simulink model "bimanual_Diedrichsen"  (Simulink 8.1)
settings: Solver=ode4  SolverMode=SingleTasking  StartTime=0.0  StopTime=inf  FixedStep=0.0005  RelTol=1e-3
StartFcn:
  |  warndlg('Dexterit-E models cannot run under simulation. Please compile your model and run it from within Dexterit-E.');set_param(bdroot,'SimulationCommand','stop')
undefined symbols (not defined in the file or in its folder): slselsubs
libraries: Video x3, General x3, KINARM_EP_loads x3, KINARM_general x2, KINARM_loads x2, xpclib x1
(part 2 of 3)

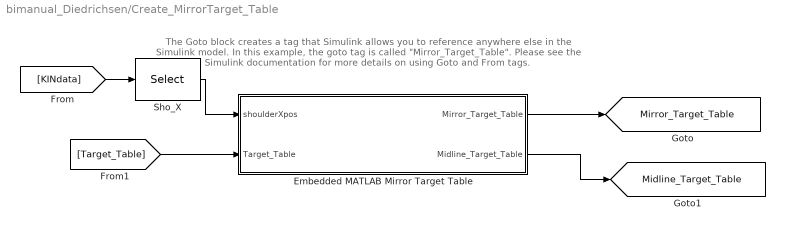
== system bimanual_Diedrichsen/Create_MirrorTarget_Table ==
  note: The Goto block creates a tag that Simulink allows you to reference anywhere else in the Simulink model.
      | In this example, the goto tag is called "Mirror_Target_Table".  Please see the Simulink documentation for more
      | details on using Goto and From tags.
  Embedded MATLAB Mirror Target Table : MATLAB Function  TreatAsAtomicUnit=on
  Sho_X : Selector  NumberOfDimensions=2  InputPortWidth=3  IndexOptions=Index vector (dialog),Index vector (dialog)  Indices=[1:2],[4]  OutputSizes=1
  tag scope: Midline_Target_Table=global, Mirror_Target_Table=global
  wires:
  [Target_Table] -> Embedded MATLAB Mirror Target Table/2(Target_Table)
  [KINdata] -> Sho_X/1
  Embedded MATLAB Mirror Target Table/1(Mirror_Target_Table) -> [Mirror_Target_Table]
  Sho_X/1 -> Embedded MATLAB Mirror Target Table/1(shoulderXpos)
  Embedded MATLAB Mirror Target Table/2(Midline_Target_Table) -> [Midline_Target_Table]

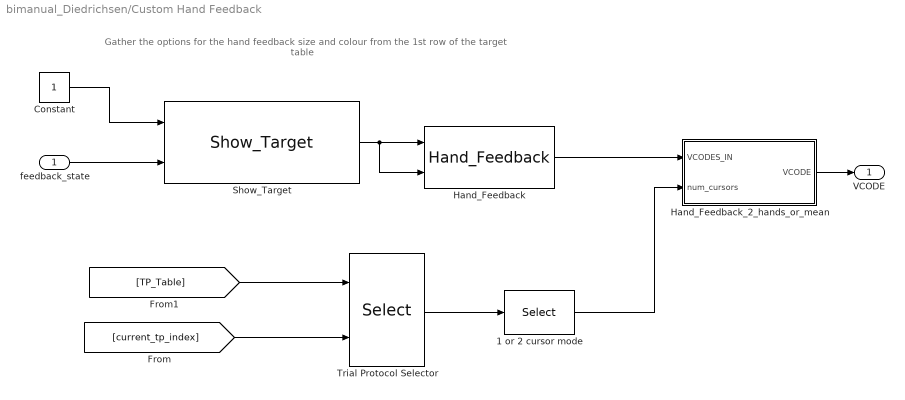
== system bimanual_Diedrichsen/Custom Hand Feedback ==
  note: Gather the options for the hand feedback size and colour from the 1st row of the target table
  "feedback_state " : Inport
  1 or 2 cursor mode : Selector  IndexOptions=Index vector (dialog)  Indices=4  OutputSizes=1
  Constant : Constant
  Hand_Feedback : KINARM_general/Hand_Feedback  feedback_cntl_src=style and status
  Hand_Feedback_2_hands_or_mean : Subsystem
  Show_Target : Video/Show_Target  target_type=Circle  num_states=4  attribcol1=[6 6 0 3]  attribcol2=[7 7 0 5]  attribcol3=[8 8 0 5]  attribcol4=[9 9 0 5]  attribcol5=[0 0 24 0]  stateindices_padding=[0 0 0 0 0 0 0;0 0 0 0 0 0 0;0 0 0 0 0 0 0;0 0 0 0 0 0 0;0 0 0 0 0 0 0]  source=dialog  opacity=100  target_display=Both subject and operator displays  num_col=4
  Trial Protocol Selector : Selector  NumberOfDimensions=2  InputPortWidth=3  IndexOptions=Index vector (port),Select all  Indices=1,-1  OutputSizes=1
  VCODE : Outport
  wires:
  "feedback_state "/1 -> Show_Target/2
  Constant/1 -> Show_Target/1
  Show_Target/1 -> Hand_Feedback/2, Hand_Feedback/1
  Trial Protocol Selector/1 -> 1 or 2 cursor mode/1
  [current_tp_index] -> Trial Protocol Selector/2
  [TP_Table] -> Trial Protocol Selector/1
  Hand_Feedback/1 -> Hand_Feedback_2_hands_or_mean/1(VCODES_IN)
  1 or 2 cursor mode/1 -> Hand_Feedback_2_hands_or_mean/2(num_cursors)
  Hand_Feedback_2_hands_or_mean/1(VCODE) -> VCODE/1

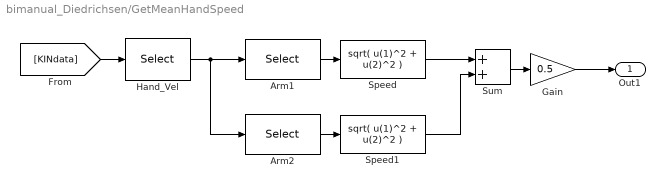
== system bimanual_Diedrichsen/GetMeanHandSpeed ==
  Arm1 : Selector  NumberOfDimensions=2  InputPortWidth=3  IndexOptions=Index vector (dialog),Select all  Indices=1,-1  OutputSizes=1
  Arm2 : Selector  NumberOfDimensions=2  InputPortWidth=3  IndexOptions=Index vector (dialog),Select all  Indices=2,-1  OutputSizes=1
  Gain : Gain  Gain=0.5
  Hand_Vel : Selector  NumberOfDimensions=2  InputPortWidth=3  IndexOptions=Select all,Index vector (dialog)  Indices=-1,[25,26]  OutputSizes=1
  Speed : Fcn  Expr=sqrt( u(1)^2 + u(2)^2 )
  Speed1 : Fcn  Expr=sqrt( u(1)^2 + u(2)^2 )
  Sum : Sum
  Out1 : Outport
  wires:
  Arm2/1 -> Speed1/1
  Sum/1 -> Gain/1
  Hand_Vel/1 -> Arm1/1, Arm2/1
  Arm1/1 -> Speed/1
  [KINdata] -> Hand_Vel/1
  Speed/1 -> Sum/1
  Speed1/1 -> Sum/2
  Gain/1 -> Out1/1

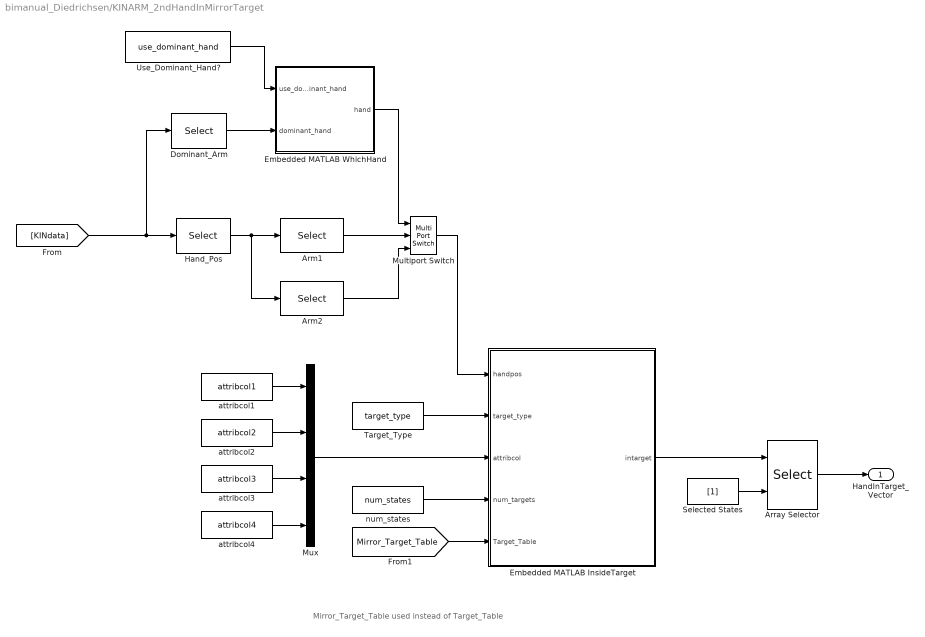
== system bimanual_Diedrichsen/KINARM_2ndHandInMirrorTarget ==
  note: Mirror_Target_Table used instead of Target_Table
  Arm1 : Selector  NumberOfDimensions=2  InputPortWidth=3  IndexOptions=Index vector (dialog),Select all  Indices=1,-1  OutputSizes=slselsubs([(-2),(-2)],1),slselsubs([(-2),(-2)],2)
  Arm2 : Selector  NumberOfDimensions=2  InputPortWidth=3  IndexOptions=Index vector (dialog),Select all  Indices=2,-1  OutputSizes=slselsubs([(-2),(-2)],1),slselsubs([(-2),(-2)],2)
  Array Selector : Selector  NumberOfDimensions=2  InputPortWidth=3  IndexOptions=Select all,Index vector (port)  Indices=-1,1  OutputSizes=slselsubs([(-2),(-2)],1),slselsubs([(-2),(-2)],2)
  Dominant_Arm : Selector  NumberOfDimensions=2  InputPortWidth=3  IndexOptions=Index vector (dialog),Index vector (dialog)  Indices=[3],[1]  OutputSizes=slselsubs([(-2),(-2)],1),slselsubs([(-2),(-2)],2)
  Embedded MATLAB InsideTarget : MATLAB Function  TreatAsAtomicUnit=on
  Embedded MATLAB WhichHand : MATLAB Function  TreatAsAtomicUnit=on
  Hand_Pos : Selector  NumberOfDimensions=2  InputPortWidth=3  IndexOptions=Select all,Index vector (dialog)  Indices=-1,[23,24]  OutputSizes=slselsubs([(-2),(-2)],1),slselsubs([(-2),(-2)],2)
  Multiport Switch : MultiPortSwitch  Inputs=2
  Mux : Mux
  Selected States : Constant  Value=[1]
  Target_Type : Constant  Value=target_type
  Use_Dominant_Hand? : Constant  Value=use_dominant_hand
  attribcol1 : Constant  Value=attribcol1
  attribcol2 : Constant  Value=attribcol2
  attribcol3 : Constant  Value=attribcol3
  attribcol4 : Constant  Value=attribcol4
  num_states : Constant  Value=num_states
  HandInTarget_Vector : Outport
  wires:
  Selected States/1 -> Array Selector/2
  num_states/1 -> Embedded MATLAB InsideTarget/4(num_targets)
  Mux/1 -> Embedded MATLAB InsideTarget/3(attribcol)
  attribcol4/1 -> Mux/4
  attribcol3/1 -> Mux/3
  attribcol2/1 -> Mux/2
  attribcol1/1 -> Mux/1
  Use_Dominant_Hand?/1 -> Embedded MATLAB WhichHand/1(use_dominant_hand)
  Embedded MATLAB WhichHand/1(hand) -> Multiport Switch/1
  Target_Type/1 -> Embedded MATLAB InsideTarget/2(target_type)
  Array Selector/1 -> HandInTarget_Vector/1
  [Mirror_Target_Table] -> Embedded MATLAB InsideTarget/5(Target_Table)
  Embedded MATLAB InsideTarget/1(intarget) -> Array Selector/1
  Multiport Switch/1 -> Embedded MATLAB InsideTarget/1(handpos)
  Arm2/1 -> Multiport Switch/3
  Arm1/1 -> Multiport Switch/2
  Dominant_Arm/1 -> Embedded MATLAB WhichHand/2(dominant_hand)
  Hand_Pos/1 -> Arm2/1, Arm1/1
  [KINdata] -> Dominant_Arm/1, Hand_Pos/1

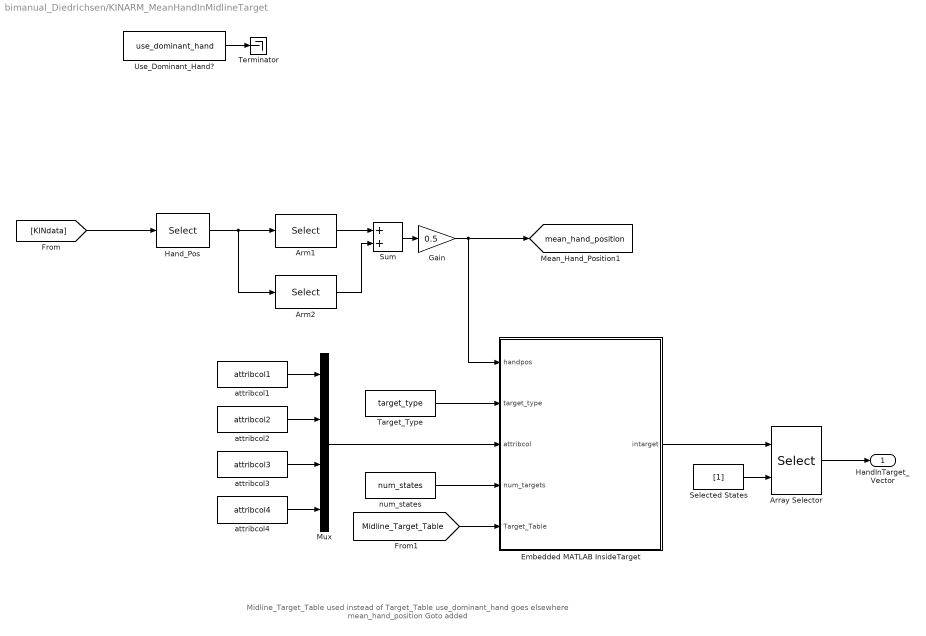
== system bimanual_Diedrichsen/KINARM_MeanHandInMidlineTarget ==
  note: Midline_Target_Table used instead of Target_Table
      | use_dominant_hand goes elsewhere
      | mean_hand_position Goto added
  Arm1 : Selector  NumberOfDimensions=2  InputPortWidth=3  IndexOptions=Index vector (dialog),Select all  Indices=1,-1  OutputSizes=1
  Arm2 : Selector  NumberOfDimensions=2  InputPortWidth=3  IndexOptions=Index vector (dialog),Select all  Indices=2,-1  OutputSizes=1
  Array Selector : Selector  NumberOfDimensions=2  InputPortWidth=3  IndexOptions=Select all,Index vector (port)  Indices=-1,1  OutputSizes=slselsubs([(-2),(-2)],1),slselsubs([(-2),(-2)],2)
  Embedded MATLAB InsideTarget : MATLAB Function  TreatAsAtomicUnit=on
  Gain : Gain  Gain=0.5
  Hand_Pos : Selector  NumberOfDimensions=2  InputPortWidth=3  IndexOptions=Select all,Index vector (dialog)  Indices=-1,[23,24]  OutputSizes=1
  Mux : Mux
  Selected States : Constant  Value=[1]
  Sum : Sum
  Target_Type : Constant  Value=target_type
  Terminator : Terminator
  Use_Dominant_Hand? : Constant  Value=use_dominant_hand
  attribcol1 : Constant  Value=attribcol1
  attribcol2 : Constant  Value=attribcol2
  attribcol3 : Constant  Value=attribcol3
  attribcol4 : Constant  Value=attribcol4
  num_states : Constant  Value=num_states
  HandInTarget_Vector : Outport
  tag scope: mean_hand_position=global
  wires:
  Selected States/1 -> Array Selector/2
  num_states/1 -> Embedded MATLAB InsideTarget/4(num_targets)
  Mux/1 -> Embedded MATLAB InsideTarget/3(attribcol)
  attribcol4/1 -> Mux/4
  attribcol3/1 -> Mux/3
  attribcol2/1 -> Mux/2
  attribcol1/1 -> Mux/1
  Target_Type/1 -> Embedded MATLAB InsideTarget/2(target_type)
  Array Selector/1 -> HandInTarget_Vector/1
  [Midline_Target_Table] -> Embedded MATLAB InsideTarget/5(Target_Table)
  Embedded MATLAB InsideTarget/1(intarget) -> Array Selector/1
  Gain/1 -> [mean_hand_position], Embedded MATLAB InsideTarget/1(handpos)
  Arm2/1 -> Sum/2
  Arm1/1 -> Sum/1
  Hand_Pos/1 -> Arm2/1, Arm1/1
  [KINdata] -> Hand_Pos/1
  Use_Dominant_Hand?/1 -> Terminator/1
  Sum/1 -> Gain/1

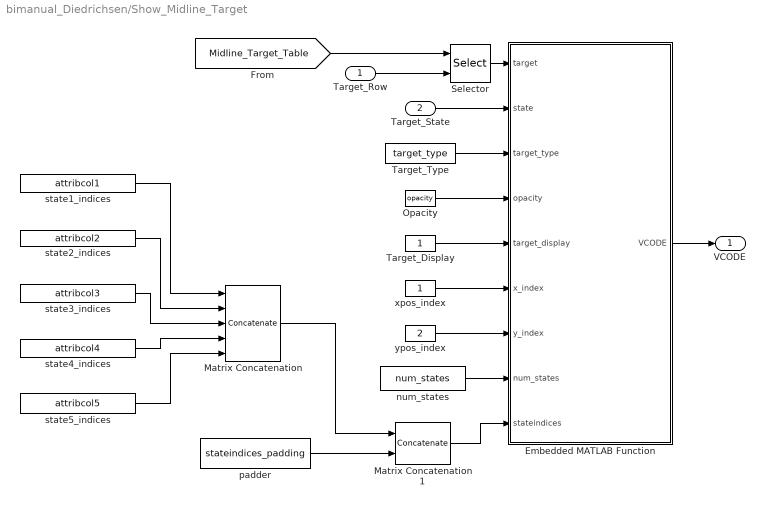
== system bimanual_Diedrichsen/Show_Midline_Target ==
  Target_Row : Inport
  Target_State : Inport  Port=2
  Embedded MATLAB Function : MATLAB Function  TreatAsAtomicUnit=on
  Matrix Concatenation : Concatenate  NumInputs=5  Mode=Multidimensional array
  Matrix Concatenation1 : Concatenate  Mode=Multidimensional array  ConcatenateDimension=2
  Opacity : Constant  Value=opacity
  Selector : Selector  NumberOfDimensions=2  InputPortWidth=3  IndexOptions=Index vector (port),Select all  Indices=1,-1  OutputSizes=slselsubs([(-2),(-2)],1),slselsubs([(-2),(-2)],2)
  Target_Display : Constant
  Target_Type : Constant  Value=target_type
  num_states : Constant  Value=num_states
  padder : Constant  Value=stateindices_padding
  state1_indices : Constant  Value=attribcol1  VectorParams1D=off
  state2_indices : Constant  Value=attribcol2  VectorParams1D=off
  state3_indices : Constant  Value=attribcol3  VectorParams1D=off
  state4_indices : Constant  Value=attribcol4  VectorParams1D=off
  state5_indices : Constant  Value=attribcol5  VectorParams1D=off
  xpos_index : Constant
  ypos_index : Constant  Value=2
  VCODE : Outport  PortDimensions=[1 70]
  wires:
  Target_Display/1 -> Embedded MATLAB Function/5(target_display)
  state2_indices/1 -> Matrix Concatenation/2
  state1_indices/1 -> Matrix Concatenation/1
  state5_indices/1 -> Matrix Concatenation/5
  state4_indices/1 -> Matrix Concatenation/4
  state3_indices/1 -> Matrix Concatenation/3
  Matrix Concatenation1/1 -> Embedded MATLAB Function/9(stateindices)
  padder/1 -> Matrix Concatenation1/2
  Matrix Concatenation/1 -> Matrix Concatenation1/1
  num_states/1 -> Embedded MATLAB Function/8(num_states)
  ypos_index/1 -> Embedded MATLAB Function/7(y_index)
  xpos_index/1 -> Embedded MATLAB Function/6(x_index)
  Target_Type/1 -> Embedded MATLAB Function/3(target_type)
  Embedded MATLAB Function/1(VCODE) -> VCODE/1
  Target_State/1 -> Embedded MATLAB Function/2(state)
  Selector/1 -> Embedded MATLAB Function/1(target)
  [Midline_Target_Table] -> Selector/1
  Target_Row/1 -> Selector/2
  Opacity/1 -> Embedded MATLAB Function/4(opacity)

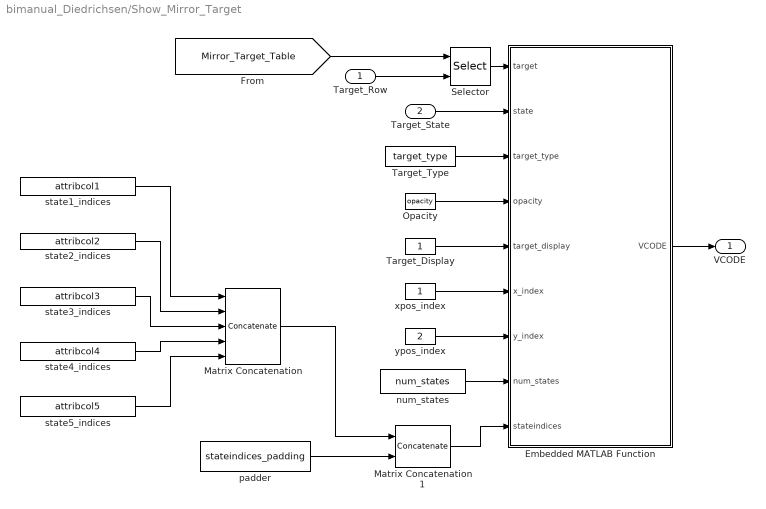
== system bimanual_Diedrichsen/Show_Mirror_Target ==
  Target_Row : Inport
  Target_State : Inport  Port=2
  Embedded MATLAB Function : MATLAB Function  TreatAsAtomicUnit=on
  Matrix Concatenation : Concatenate  NumInputs=5  Mode=Multidimensional array
  Matrix Concatenation1 : Concatenate  Mode=Multidimensional array  ConcatenateDimension=2
  Opacity : Constant  Value=opacity
  Selector : Selector  NumberOfDimensions=2  InputPortWidth=3  IndexOptions=Index vector (port),Select all  Indices=1,-1  OutputSizes=slselsubs([(-2),(-2)],1),slselsubs([(-2),(-2)],2)
  Target_Display : Constant
  Target_Type : Constant  Value=target_type
  num_states : Constant  Value=num_states
  padder : Constant  Value=stateindices_padding
  state1_indices : Constant  Value=attribcol1  VectorParams1D=off
  state2_indices : Constant  Value=attribcol2  VectorParams1D=off
  state3_indices : Constant  Value=attribcol3  VectorParams1D=off
  state4_indices : Constant  Value=attribcol4  VectorParams1D=off
  state5_indices : Constant  Value=attribcol5  VectorParams1D=off
  xpos_index : Constant
  ypos_index : Constant  Value=2
  VCODE : Outport  PortDimensions=[1 70]
  wires:
  Target_Display/1 -> Embedded MATLAB Function/5(target_display)
  state2_indices/1 -> Matrix Concatenation/2
  state1_indices/1 -> Matrix Concatenation/1
  state5_indices/1 -> Matrix Concatenation/5
  state4_indices/1 -> Matrix Concatenation/4
  state3_indices/1 -> Matrix Concatenation/3
  Matrix Concatenation1/1 -> Embedded MATLAB Function/9(stateindices)
  padder/1 -> Matrix Concatenation1/2
  Matrix Concatenation/1 -> Matrix Concatenation1/1
  num_states/1 -> Embedded MATLAB Function/8(num_states)
  ypos_index/1 -> Embedded MATLAB Function/7(y_index)
  xpos_index/1 -> Embedded MATLAB Function/6(x_index)
  Target_Type/1 -> Embedded MATLAB Function/3(target_type)
  Embedded MATLAB Function/1(VCODE) -> VCODE/1
  Target_State/1 -> Embedded MATLAB Function/2(state)
  Selector/1 -> Embedded MATLAB Function/1(target)
  [Mirror_Target_Table] -> Selector/1
  Target_Row/1 -> Selector/2
  Opacity/1 -> Embedded MATLAB Function/4(opacity)

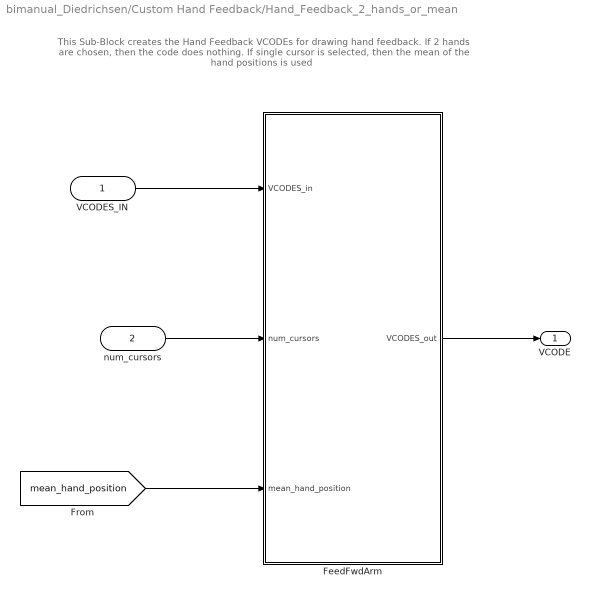
== system bimanual_Diedrichsen/Custom Hand Feedback/Hand_Feedback_2_hands_or_mean ==
  note: This Sub-Block creates the Hand Feedback VCODEs for drawing hand feedback.
      | If 2 hands are chosen, then the code does nothing. If single cursor is selected, then the mean of the hand positions is used
  VCODES_IN : Inport
  num_cursors : Inport  Port=2
  FeedFwdArm : MATLAB Function  TreatAsAtomicUnit=on
  VCODE : Outport
  wires:
  FeedFwdArm/1(VCODES_out) -> VCODE/1
  VCODES_IN/1 -> FeedFwdArm/1(VCODES_in)
  num_cursors/1 -> FeedFwdArm/2(num_cursors)
  [mean_hand_position] -> FeedFwdArm/3(mean_hand_position)

== stateflow chart Trial_Control ==
  settings: sampleTime=0.001
  state Inter_Trial_State/
    // send e_Trial_End event
    e_Trial_End;
    // reset event_code
    event_code=0;
    // turn off both targets
    targetA_state=0;
    targetB_state=0;
    // stop data logging
    logging_enable = 0;
    // turn on hand feedback
    hand_feedback = 1;
  state Main_Trial
    state Show2ndTargets/
      // Move targets to second target position(s), log an event,
      // Then wait until either mean hand speed goes reaches below threshold or for specified delay
      event_code=E_TARGET_ON;
      target_row = Trial_Protocol[COL_END_TARGET];
      tickCount =2000;
    state StayAt2ndTarget/
      // log an event, wait for a specified period of time
      event_code = E_HOLD_AT_TARGET;
      tickCount = Trial_Protocol[COL_2ND_TARGET_WAIT];
    state EndOfTrial/
      // Wait for a specified period of time,
      tickCount =Trial_Protocol[COL_POST_TRIAL_DELAY];
    state StayAtFirstTargets/
      // log an event, Hand must STAY in target for specified time before trial proceeds.
      logging_enable = 1;
      event_code=E_STAY_CENTER;
    state WaitForMovementEnds/
      // Movement has started (i.e. speed > 3 cm/s), wait for
      // movement end (i.e. speed < 1.5 cm/s)
      tickCount2=Trial_Protocol[COL_MAX_REACH_TIME]
    state WaitForHandToReachMeanTarget/
      // mean hand position (i.e. as shown to subject)
      //must be in target
    state TooSlow/
    state WaitForHandsToReachFirstTargets/
      // Both hands must be in their respective targets
    state StayAtFirstTarget/
      // log an event, Hand must STAY in target for specified time before trial proceeds.
      logging_enable = 1;
      event_code=E_STAY_CENTER;
    (junction 15) -> (junction 16) : // Initialize the trial conditions
        | /
        | target_row = Trial_Protocol[COL_START_TARGET];
        | load_row = Trial_Protocol[COL_LOAD];
        | tickCount =Trial_Protocol[COL_1ST_TARGET_WAIT]+Trial_Protocol[COL_RANDOM_WAIT]*rand()/RAND_MAX;
    (junction 16) -> WaitForHandsToReachFirstTargets [order 1] : [Trial_Protocol[COL_CURSOR_SELECTION]==2]/
        | targetA_state=1;
        | // If the trial protocol requests two targets, one for each arm, then
        | // proceed down this logid and turn on initial targets
    (junction 16) -> WaitForHandToReachMeanTarget [order 2] : /
        | // Otherwise proceed down this logid and turn on initial target
        | targetB_state=1;
    StayAtFirstTargets -> WaitForHandsToReachFirstTargets [order 2] : [HandInTarget[target_row]==0 || HandIn2ndTarget[target_row]==0]
    WaitForHandToReachMeanTarget -> StayAtFirstTarget : [HandMeanInTarget[target_row]==1]
    StayAtFirstTarget -> WaitForHandToReachMeanTarget [order 2] : [HandMeanInTarget[target_row]==0]
    WaitForHandsToReachFirstTargets -> StayAtFirstTargets : [HandInTarget[target_row]==1 && HandIn2ndTarget[target_row]==1]
    StayAtFirstTargets -> Show2ndTargets [order 1] : after(tickCount, e_clk)
    StayAtFirstTarget -> Show2ndTargets [order 1] : after(tickCount, e_clk)
    Show2ndTargets -> (junction 17) [order 2] : [MeanHandSpeed > SPEEDTHRESHOLDSTART]
    Show2ndTargets -> StayAt2ndTarget [order 1] : after(tickCount, e_clk)/
        | hand_feedback=3
        | //too slow
    (junction 17) -> WaitForMovementEnds [order 1] : [Trial_Protocol[COL_HAND_FEEDBACK]==0]/
        | hand_feedback=0;
        | // log an event that hand feedback is now off
        | event_code=E_HAND_FDBK_OFF;
    (junction 17) -> WaitForMovementEnds [order 2]
    WaitForMovementEnds -> TooSlow [order 1] : after(tickCount2, e_clk)
    WaitForMovementEnds -> (junction 18) [order 2] : [MeanHandSpeed < SPEEDTHRESHOLDSTOP]
    (junction 18) -> StayAt2ndTarget [order 1] : [(Trial_Protocol[COL_CURSOR_SELECTION]==2 && HandInTarget[target_row]==1 && HandIn2ndTarget[target_row]==1) ...
        | || (Trial_Protocol[COL_CURSOR_SELECTION]==1 && HandMeanInTarget[target_row]==1)]/
        | hand_feedback=2;
        | // Change hand feedback colour to indicate to subject a "good" movement
    (junction 18) -> StayAt2ndTarget [order 2] : /
        | hand_feedback=4;
        | // Change hand feedback colour to indicate to
        | // subject that they missed the targets
    TooSlow -> StayAt2ndTarget : [MeanHandSpeed < SPEEDTHRESHOLDSTOP]/
        | hand_feedback=3;
        | // Change hand feedback colour to indicate to subject that they were too "slow"
    StayAt2ndTarget -> EndOfTrial : after(tickCount, e_clk)
  state Initialize/
    // Turn off both targets, turn off any loads and
    // set hand_feedback on
    targetA_state=0;
    targetB_state=0;
    hand_feedback = 1;
  (default) -> Initialize
  Initialize -> (junction 15)
  Inter_Trial_State -> (junction 15) : after(tickCount, e_clk)
  Main_Trial -> Inter_Trial_State : e_ExitTrialNow/
      | // if e_ExitTrialNow event occurs,
      | tickCount=1;
  EndOfTrial -> Inter_Trial_State
  data: logging_enable output boolean; HandInTarget input double; event_code output uint16 [0..] =4101; load_row output double [1..32]; target_row output double [1..32]; targetA_state output double; targetB_state output double; tickCount local double; hand_feedback output double; HandIn2ndTarget input double; HandMeanInTarget input double; MeanHandSpeed input double; Trial_Protocol input double; tickCount2 local double; SPEEDTHRESHOLDSTART constant double =0.03; SPEEDTHRESHOLDSTOP constant double =0.015; RAND_MAX constant double =32767
  data load_row settings: description=current index into the loadtable
  data target_row settings: description=index of the row currently being used in the TargetTable
  events: e_clk input RISING_EDGE_EVENT; e_ExitTrialNow input EITHER_EDGE_EVENT; e_Trial_End output EITHER_EDGE_EVENT

== matlab function KINARM_2ndHandInMirrorTarget/Embedded MATLAB InsideTarget ==
  settings: fimath=|
      | fimath(...
      | 'RoundMode', 'floor',...
      | 'OverflowMode', 'wrap',...
      | 'ProductMode', 'KeepLSB', 'ProductWordLength', 32,...
      | 'SumMode', 'KeepLSB', 'SumWordLength', 32,...
      | 'CastBeforeSum', false)
  data: handpos input double size=2; target_type input double; attribcol input double; num_targets input double; intarget output double; Target_Table input double
function intarget = FIsInsideTarget(handpos, target_type, attribcol, num_targets, Target_Table)
% all dimensions in m, rad
% arguments:
% handpos: x,y positions of center of target
% attribcol: columns in target table specifying target attributes.  
% Specific to Target_Type
%	circle:
%	[X0,Y0,r...,rn] where:
%	X0,Y0 : centre of circle
%	r : logical radius of circle (i.e. radius used to determine 'in' or 'out' of target)
%	rn: logical radius of other targets (e.g. 2nd, 3rd) also specified in target row.
%   Up to 4 targets can be specified in a row
% ellipse:
%	[X0,Y0,a,b,t...,an, bn, tn] where:
%	X0,Y0 : centre of ellipse
%	a,b : major, minor radii of ellipse
%	t : rotation of ellipse in degrees
%	an,bn : major, minor radii of ellipse of other targets (e.g. 2nd, 3rd) also specified in target row
%	tn : rotation of ellipse in degrees of other targets (e.g. 2nd, 3rd) also specified in target row
%   Up to 4 targets can be specified in a row


target_col_x=1;
target_col_y=2;

x=handpos(1);
y=handpos(2);

intarget = zeros(size(Target_Table,1),4);

X0 = Target_Table(:,target_col_x)*0.01;			%Target Table sizes in cm in v1.4
Y0 = Target_Table(:,target_col_y)*0.01;			%Target Table sizes in cm in v1.4

deltax=x-X0;
deltay=y-Y0;

INT_MAX=2^32-1;

if target_type==1			%circle
	for target=1:num_targets
		r = Target_Table(:,attribcol(target))*0.01;			%Target Table sizes in cm in v1.4
		% simple euclidean distance
		distance2 = deltax.^2 + deltay.^2;					%distance2 is the square of the distance
	    intarget(:,target) = (distance2 <= r.^2);
	end
elseif target_type==2		%ellipse
	for target=1:num_targets
	    a = Target_Table(:,attribcol(target*3-2))*0.01;			%Target Table sizes in cm in v1.4
	    b = Target_Table(:,attribcol(target*3-1))*0.01;			%Target Table sizes in cm in v1.4	
	    t = Target_Table(:,attribcol(target*3))*(pi / 180.0);	%Target Table angles in degrees in v1.4
		sint=sin(t);
		cost=cos(t);
		xrotate=deltax.*cost+deltay.*sint;		%location of x point in ellipse's coordinate frame
		yrotate=-deltax.*sint+deltay.*cost;		%location of y point in ellipse's coordinate frame
		m=yrotate./xrotate;						%slope of line between the (x,y) to (x0,y0) in ellipse's coordinate frame
		y2sq=1./(1./(m.*a).^2+1./b.^2);			%y2sq is y2^2, where y2 is the intersection of the ellipse and the (x,y) to (x0,y0) line
	    intarget(:,target) = (yrotate.^2 <= y2sq);
    end
elseif target_type==3       %rectangle
    for target=1:num_targets
        w = Target_Table(:,attribcol(target*3-2))*0.01;  %width (sizes in cm in v1.4)
        h = Target_Table(:,attribcol(target*3-1))*0.01;  %height (sizes in cm in v1.4)
        
        if attribcol(target*3) > 0
            t = Target_Table(:,attribcol(target*3))*(pi / 180.0);  %angle (angles in degrees in v1.4)
        else
            t = zeros(size(Target_Table, 1), 1);
        end

        sint=sin(t);
        cost=cos(t);

        xrotate=deltax.*cost + deltay.*sint;   %location of x point in rectangle's coordinate frame
        yrotate=-deltax.*sint + deltay.*cost;  %location of y point in rectangle's coordinate frame

        intarget(:,target) = abs(xrotate) <= w/2 & abs(yrotate) <= h/2;
    end
elseif target_type==4       %line
    for target=1:num_targets
        % treat the line like a rectangle of height h and width w
        % determine height (stroke width) in the same fashion as in Show_Target
        if attribcol(target*3-2) == 0                     %0 column index means stroke width of 0
            h = zeros(size(Target_Table, 1), 1);
        elseif attribcol(target*3-2) < 0                  %-ve column index means stroke width of 1mm
            h = ones(size(Target_Table, 1), 1) .* 0.001;
        else
            h = Target_Table(:,attribcol(target*3-2)) * 0.01;  %target table contains width in cm
        end
        
        ex = Target_Table(:,attribcol(target*3-1))*0.01;  %endpoint in x relative to start point (cm)
        ey = Target_Table(:,attribcol(target*3))*0.01;    %endpoint in y relative to start point (cm)
        
        w = sqrt(ex.^2 + ey.^2);                          %width (cm)
        
        % determine the vector from the line's midpoint to the hand position
        handx = deltax - ex/2;
        handy = deltay - ey/2;
        
        t = atan2(ey, ex);                                %calculate angle of the line (rads)
        sint = sin(t);
        cost = cos(t);
        
        xrotate = handx.*cost + handy.*sint;   %location of x point in rectangle's coordinate frame
        yrotate = -handx.*sint + handy.*cost;  %location of y point in rectangle's coordinate frame
 
        intarget(:,target) = abs(xrotate) <= w/2 & abs(yrotate) <= h/2;
    end
elseif target_type==5  % triangle
    for target=1:num_targets
        w = Target_Table(:,attribcol(target*4-3))*0.01;         %length (sizes in cm in v1.4)
        
        % If a height column of 0 is specified, make the triangle equilateral. Otherwise, use the
        % values for height and peak offset from the target table.
        if attribcol(target*4-2) > 0
            h = Target_Table(:,attribcol(target*4-2))*0.01;  %height (sizes in cm in v1.4)
            p = Target_Table(:,attribcol(target*4-1))*0.01;  %peak offset (sizes in cm in v1.4)
        else
            h = w.*sin(pi/3.0);
            p = zeros(size(Target_Table, 1), 1);
        end
        
        if attribcol(target*4) > 0
            t = Target_Table(:,attribcol(target*4))*(pi / 180.0);  %angle (angles in degrees in v1.4)
        else
            t = zeros(size(Target_Table, 1), 1);
        end
        
        sint = sin(t);
        cost = cos(t);
        
        xrotate = deltax.*cost + deltay.*sint;   %location of x point in triangle's coordinate frame
        yrotate = -deltax.*sint + deltay.*cost;  %location of y point in triangle's coordinate frame
        
        % Begin to find centroid of triangle relative to the point on the base beneath the peak. "Left vertex" 
        % refers to the vertex at the left end of the base, and "right vertex" to the vertex at the right end.
        n = w./2.0 + p;  % distance along base from left vertex to peak
        m = w./2.0 - p;  % distance along base from peak to right vertex

        alpha = atan2(h, n);  % angle between base and line from left vertex to peak
        beta = atan2(h, m);   % angle between base and line from right vertex to peak
        
        length1 = sqrt(h.*h + n.*n) ./ 2.0;  % half length of line from left vertex to peak
        length2 = sqrt(h.*h + m.*m) ./ 2.0;  % half length of line from right vertex to peak

        % Determine slope of line from left vertex to midpoint of line from right vertex to peak.
        slope1 = ones(size(Target_Table, 1), 1) .* INT_MAX;
        
        for i=1:size(Target_Table, 1)
            if abs(w(i) - length2(i)*cos(beta(i))) > 0.0
                slope1(i) = length2(i)*sin(beta(i)) / (w(i) - length2(i)*cos(beta(i)));
            end
        end

        % Determine slope of line from right vertex to midpoint of line from left vertex to peak.
        slope2 = ones(size(Target_Table, 1), 1) .* INT_MAX;

        for i=1:size(Target_Table, 1)
            if abs(w(i) - length1(i)*cos(alpha(i))) > 0.0
                slope2(i) = -length1(i)*sin(alpha(i)) / (w(i) - length1(i)*cos(alpha(i)));
            end
        end

        % Calculate centroid position.
        centroid_x = -(m.*slope2 + n.*slope1) ./ (slope1 - slope2);
        centroid_y = slope1.*(centroid_x + n);

        % Test if the point is under the left side of the peak.
        is_under_left = false(size(Target_Table, 1), 1);

        for i=1:size(Target_Table, 1)
            if n(i) >= 0
                is_under_left(i) = (h(i) + (h(i)/n(i)) * (xrotate(i) + centroid_x(i))) >= (yrotate(i) + centroid_y(i));
            else
                is_under_left(i) = (h(i) + (h(i)/n(i)) * (xrotate(i) + centroid_x(i))) <= (yrotate(i) + centroid_y(i));
            end
        end
        
        % Test if the point is under the right side of the peak.
        is_under_right = false(size(Target_Table, 1), 1);

        for i=1:size(Target_Table, 1)
            if m(i) >= 0
                is_under_right(i) = (h(i) - (h(i)/m(i)) * (xrotate(i) + centroid_x(i))) >= (yrotate(i) + centroid_y(i));
            else
                is_under_right(i) = (h(i) - (h(i)/m(i)) * (xrotate(i) + centroid_x(i))) <= (yrotate(i) + centroid_y(i));
            end
        end
        
        intarget(:,target) = is_under_right & ...            %under right side of peak
                             is_under_left & ...             %under left side of peak
                             (yrotate + centroid_y) >= 0.0;  %above base
    end
end

== matlab function KINARM_MeanHandInMidlineTarget/Embedded MATLAB InsideTarget ==
  settings: fimath=|
      | fimath(...
      | 'RoundMode', 'floor',...
      | 'OverflowMode', 'wrap',...
      | 'ProductMode', 'KeepLSB', 'ProductWordLength', 32,...
      | 'SumMode', 'KeepLSB', 'SumWordLength', 32,...
      | 'CastBeforeSum', false)
  data: handpos input double size=2; target_type input double; attribcol input double; num_targets input double; intarget output double; Target_Table input double
function intarget = FIsInsideTarget(handpos, target_type, attribcol, num_targets, Target_Table)
% all dimensions in m, rad
% arguments:
% handpos: x,y positions of center of target
% attribcol: columns in target table specifying target attributes.  
% Specific to Target_Type
%	circle:
%	[X0,Y0,r...,rn] where:
%	X0,Y0 : centre of circle
%	r : logical radius of circle (i.e. radius used to determine 'in' or 'out' of target)
%	rn: logical radius of other targets (e.g. 2nd, 3rd) also specified in target row.
%   Up to 4 targets can be specified in a row
% ellipse:
%	[X0,Y0,a,b,t...,an, bn, tn] where:
%	X0,Y0 : centre of ellipse
%	a,b : major, minor radii of ellipse
%	t : rotation of ellipse in degrees
%	an,bn : major, minor radii of ellipse of other targets (e.g. 2nd, 3rd) also specified in target row
%	tn : rotation of ellipse in degrees of other targets (e.g. 2nd, 3rd) also specified in target row
%   Up to 4 targets can be specified in a row


target_col_x=1;
target_col_y=2;

x=handpos(1);
y=handpos(2);

intarget = zeros(size(Target_Table,1),4);

X0 = Target_Table(:,target_col_x)*0.01;			%Target Table sizes in cm in v1.4
Y0 = Target_Table(:,target_col_y)*0.01;			%Target Table sizes in cm in v1.4

deltax=x-X0;
deltay=y-Y0;

INT_MAX=2^32-1;

if target_type==1			%circle
	for target=1:num_targets
		r = Target_Table(:,attribcol(target))*0.01;			%Target Table sizes in cm in v1.4
		% simple euclidean distance
		distance2 = deltax.^2 + deltay.^2;					%distance2 is the square of the distance
	    intarget(:,target) = (distance2 <= r.^2);
	end
elseif target_type==2		%ellipse
	for target=1:num_targets
	    a = Target_Table(:,attribcol(target*3-2))*0.01;			%Target Table sizes in cm in v1.4
	    b = Target_Table(:,attribcol(target*3-1))*0.01;			%Target Table sizes in cm in v1.4	
	    t = Target_Table(:,attribcol(target*3))*(pi / 180.0);	%Target Table angles in degrees in v1.4
		sint=sin(t);
		cost=cos(t);
		xrotate=deltax.*cost+deltay.*sint;		%location of x point in ellipse's coordinate frame
		yrotate=-deltax.*sint+deltay.*cost;		%location of y point in ellipse's coordinate frame
		m=yrotate./xrotate;						%slope of line between the (x,y) to (x0,y0) in ellipse's coordinate frame
		y2sq=1./(1./(m.*a).^2+1./b.^2);			%y2sq is y2^2, where y2 is the intersection of the ellipse and the (x,y) to (x0,y0) line
	    intarget(:,target) = (yrotate.^2 <= y2sq);
    end
elseif target_type==3       %rectangle
    for target=1:num_targets
        w = Target_Table(:,attribcol(target*3-2))*0.01;  %width (sizes in cm in v1.4)
        h = Target_Table(:,attribcol(target*3-1))*0.01;  %height (sizes in cm in v1.4)
        
        if attribcol(target*3) > 0
            t = Target_Table(:,attribcol(target*3))*(pi / 180.0);  %angle (angles in degrees in v1.4)
        else
            t = zeros(size(Target_Table, 1), 1);
        end

        sint=sin(t);
        cost=cos(t);

        xrotate=deltax.*cost + deltay.*sint;   %location of x point in rectangle's coordinate frame
        yrotate=-deltax.*sint + deltay.*cost;  %location of y point in rectangle's coordinate frame

        intarget(:,target) = abs(xrotate) <= w/2 & abs(yrotate) <= h/2;
    end
elseif target_type==4       %line
    for target=1:num_targets
        % treat the line like a rectangle of height h and width w
        % determine height (stroke width) in the same fashion as in Show_Target
        if attribcol(target*3-2) == 0                     %0 column index means stroke width of 0
            h = zeros(size(Target_Table, 1), 1);
        elseif attribcol(target*3-2) < 0                  %-ve column index means stroke width of 1mm
            h = ones(size(Target_Table, 1), 1) .* 0.001;
        else
            h = Target_Table(:,attribcol(target*3-2)) * 0.01;  %target table contains width in cm
        end
        
        ex = Target_Table(:,attribcol(target*3-1))*0.01;  %endpoint in x relative to start point (cm)
        ey = Target_Table(:,attribcol(target*3))*0.01;    %endpoint in y relative to start point (cm)
        
        w = sqrt(ex.^2 + ey.^2);                          %width (cm)
        
        % determine the vector from the line's midpoint to the hand position
        handx = deltax - ex/2;
        handy = deltay - ey/2;
        
        t = atan2(ey, ex);                                %calculate angle of the line (rads)
        sint = sin(t);
        cost = cos(t);
        
        xrotate = handx.*cost + handy.*sint;   %location of x point in rectangle's coordinate frame
        yrotate = -handx.*sint + handy.*cost;  %location of y point in rectangle's coordinate frame
 
        intarget(:,target) = abs(xrotate) <= w/2 & abs(yrotate) <= h/2;
    end
elseif target_type==5  % triangle
    for target=1:num_targets
        w = Target_Table(:,attribcol(target*4-3))*0.01;         %length (sizes in cm in v1.4)
        
        % If a height column of 0 is specified, make the triangle equilateral. Otherwise, use the
        % values for height and peak offset from the target table.
        if attribcol(target*4-2) > 0
            h = Target_Table(:,attribcol(target*4-2))*0.01;  %height (sizes in cm in v1.4)
            p = Target_Table(:,attribcol(target*4-1))*0.01;  %peak offset (sizes in cm in v1.4)
        else
            h = w.*sin(pi/3.0);
            p = zeros(size(Target_Table, 1), 1);
        end
        
        if attribcol(target*4) > 0
            t = Target_Table(:,attribcol(target*4))*(pi / 180.0);  %angle (angles in degrees in v1.4)
        else
            t = zeros(size(Target_Table, 1), 1);
        end
        
        sint = sin(t);
        cost = cos(t);
        
        xrotate = deltax.*cost + deltay.*sint;   %location of x point in triangle's coordinate frame
        yrotate = -deltax.*sint + deltay.*cost;  %location of y point in triangle's coordinate frame
        
        % Begin to find centroid of triangle relative to the point on the base beneath the peak. "Left vertex" 
        % refers to the vertex at the left end of the base, and "right vertex" to the vertex at the right end.
        n = w./2.0 + p;  % distance along base from left vertex to peak
        m = w./2.0 - p;  % distance along base from peak to right vertex

        alpha = atan2(h, n);  % angle between base and line from left vertex to peak
        beta = atan2(h, m);   % angle between base and line from right vertex to peak
        
        length1 = sqrt(h.*h + n.*n) ./ 2.0;  % half length of line from left vertex to peak
        length2 = sqrt(h.*h + m.*m) ./ 2.0;  % half length of line from right vertex to peak

        % Determine slope of line from left vertex to midpoint of line from right vertex to peak.
        slope1 = ones(size(Target_Table, 1), 1) .* INT_MAX;
        
        for i=1:size(Target_Table, 1)
            if abs(w(i) - length2(i)*cos(beta(i))) > 0.0
                slope1(i) = length2(i)*sin(beta(i)) / (w(i) - length2(i)*cos(beta(i)));
            end
        end

        % Determine slope of line from right vertex to midpoint of line from left vertex to peak.
        slope2 = ones(size(Target_Table, 1), 1) .* INT_MAX;

        for i=1:size(Target_Table, 1)
            if abs(w(i) - length1(i)*cos(alpha(i))) > 0.0
                slope2(i) = -length1(i)*sin(alpha(i)) / (w(i) - length1(i)*cos(alpha(i)));
            end
        end

        % Calculate centroid position.
        centroid_x = -(m.*slope2 + n.*slope1) ./ (slope1 - slope2);
        centroid_y = slope1.*(centroid_x + n);

        % Test if the point is under the left side of the peak.
        is_under_left = false(size(Target_Table, 1), 1);

        for i=1:size(Target_Table, 1)
            if n(i) >= 0
                is_under_left(i) = (h(i) + (h(i)/n(i)) * (xrotate(i) + centroid_x(i))) >= (yrotate(i) + centroid_y(i));
            else
                is_under_left(i) = (h(i) + (h(i)/n(i)) * (xrotate(i) + centroid_x(i))) <= (yrotate(i) + centroid_y(i));
            end
        end
        
        % Test if the point is under the right side of the peak.
        is_under_right = false(size(Target_Table, 1), 1);

        for i=1:size(Target_Table, 1)
            if m(i) >= 0
                is_under_right(i) = (h(i) - (h(i)/m(i)) * (xrotate(i) + centroid_x(i))) >= (yrotate(i) + centroid_y(i));
            else
                is_under_right(i) = (h(i) - (h(i)/m(i)) * (xrotate(i) + centroid_x(i))) <= (yrotate(i) + centroid_y(i));
            end
        end
        
        intarget(:,target) = is_under_right & ...            %under right side of peak
                             is_under_left & ...             %under left side of peak
                             (yrotate + centroid_y) >= 0.0;  %above base
    end
end

== matlab function Create_MirrorTarget_Table/Embedded MATLAB Mirror Target Table ==
  settings: fimath=|
      | fimath(...
      | 'RoundMode', 'floor',...
      | 'OverflowMode', 'wrap',...
      | 'ProductMode', 'KeepLSB', 'ProductWordLength', 32,...
      | 'SumMode', 'KeepLSB', 'SumWordLength', 32,...
      | 'CastBeforeSum', false)
  data: shoulderXpos input double size=2; Mirror_Target_Table output double; Target_Table input double; Midline_Target_Table output double
function [Mirror_Target_Table,Midline_Target_Table]= FMirror_TT(shoulderXpos, Target_Table)
% this function creates a Mirror_Target_Table that is the mirror image of 
% the Target Table, flipped in the X-direction around the subject's midline
% The subject's midline is assumed to be halfway between the two shoulders.

% It also creates a midline Target Table with all targets on the midline.

% all dimensions in m unless otherwise stated
% arguments:
% shoulderXpos: x positions of shoulders (m)
% Target_Table: the complete Target_Table (cm in v1.4)


target_col_x = 1;
center_x = mean(shoulderXpos)*100;				%calculate the subject's midline position (cm)
Mirror_Target_Table = Target_Table;
Midline_Target_Table = Target_Table;

Mirror_Target_Table(:,target_col_x) = 2*center_x-Target_Table(:,target_col_x);
Midline_Target_Table(:,target_col_x) = center_x;

== matlab function Show_Midline_Target/Embedded MATLAB Function ==
  settings: fimath=|
      | fimath(...
      | 'RoundMode', 'floor',...
      | 'OverflowMode', 'wrap',...
      | 'ProductMode', 'KeepLSB', 'ProductWordLength', 32,...
      | 'SumMode', 'KeepLSB', 'SumWordLength', 32,...
      | 'CastBeforeSum', false)
  data: target input double; VCODE output double; state input double; target_type input double; opacity input double; target_display input double; x_index input double; y_index input double; num_states input double; stateindices input double
function VCODE  = fcn(target, state, target_type, opacity, target_display, x_index, y_index, num_states, stateindices)

% VCODEs are length 70. All units in a VCODE should be SI, e.g. (m) and (rad). Elements in a VCODE are defined as follows:
%
% For all target types:
%  1: target type
%       1 - circle
%       2 - ellipse
%       3 - rectangle
%       4 - line
%       5 - triangle
%       11 - circle with label
%       12 - ellipse with label
%       13 - rectangle with label
%       14 - line with label
%       15 - triangle with label
%  2: target on/off status and target display (which display target will appear on)
%		0 - off
%		1 - on, appearing on both subject and operator displays
%       2 - on, appearing on subject display only
%       3 - on, appearing on operator display only
%  3: x position (m)
%  4: y position (m)
%  5: fill colour (RRGGBB) or texture index
%  6: stroke colour (RRGGBB) or texture index
%  7: stroke width
%  8: reserved for target background ID
%  9: opacity
%
% For circles:
%  10: radius (m)
%
% For ellipses:
%  10: major radius (m)
%  11: minor radius (m)
%  12: orientation of major axis (rad)
%
% For rectangles:
%  10: length (m)
%  11: height (m)
%  12: orientation (rad) (relative to x, y already shown)
%
% For lines:
%  10: endpoint x-axis coordinate relative to start point (m)
%  11: endpoint y-axis coordinate relative to start point (m)
%
% For triangles:
%  10: length (m)
%  11: height (m)
%  12: offset of peak from midpoint of length (m)
%  13: orientation (rad)
%
% For all labelled target types:
%  14: reserved
%  15-64: label characters (indexes in ISO 8859-1 character set)
%  65: label colour (0xRRGGBB), opacity is set by the vcode's opacity (9).
%  66: label height (m)
%  67: reserved
%  68: reserved
%  69: reserved
%  70: reserved

VCODE = zeros(1, 70);

% Set the target type.
VCODE(1) = target_type;

% Set the target on/off state. If the state input is 0, the target is off. Users of the VCODE should respect this
% as an indication that the rest of the VCODE will be uninitialized.
if (state <= 0) || (state > num_states)
	VCODE(2) = 0;  % target is off
	return;
else
	VCODE(2) = target_display;  % target is on; target displays as specified by block mask
end

% Set the target position.
VCODE(3) = target(x_index) * 0.01;  % x position (convert from (cm) in target table to (m))
VCODE(4) = target(y_index) * 0.01;  % y position (convert from (cm) in target table to (m))

% Set the fill colour. Fill colour currently comes from the GUI in RRRGGGBBB format.
if stateindices(state, 1) == 0
	VCODE(5) = -2^31;
elseif target(stateindices(state, 1)) < 0
    VCODE(5) = target(stateindices(state, 1));
else
	VCODE(5) = colourshift(target(stateindices(state, 1)));
end

% Set the stroke colour. Stroke colour currently comes from the GUI in RRRGGGBBB format.
if stateindices(state, 2) == 0
	VCODE(6) = -2^31;
elseif target(stateindices(state, 2)) < 0
    VCODE(6) = target(stateindices(state, 2));
else
	VCODE(6) = colourshift(target(stateindices(state, 2)));
end

% Set the stroke width. if target table index for stroke width is zero, then the stroke width is undefined
if stateindices(state, 3) == 0
	VCODE(7) = 0;                   % if stroke width column is 0, then stroke width is 0
elseif stateindices(state, 3) < 0
	VCODE(7) = 0.001;               % if stroke width column is -ve, then a 1mm default is chosen
else
	VCODE(7) = target(stateindices(state, 3)) * 0.01;  % if stroke width column is +ve, convert width from (cm) in target table to (m)
end

% Set the opacity value, clamping it to [0, 100].
if opacity <= 0
    VCODE(9) = 0.0;
elseif opacity >= 100
    VCODE(9) = 100.0;
else
    VCODE(9) = opacity;
end

% Set attributes specific to each target type.
if target_type == 1

    % Handle circle target:
	VCODE(10)=target(stateindices(state, 4)) * 0.01;  % radius (convert from (cm) in target table to (m))

elseif target_type == 2

    % Handle ellipse target:
	VCODE(10) = target(stateindices(state, 4)) * 0.01;  % major radius (convert from (cm) in target table to (m))
	VCODE(11) = target(stateindices(state, 5)) * 0.01;  % minor radius (convert from (cm) in target table to (m))

    if stateindices(state, 6) == 0
		VCODE(12) = 0;  % if orientation column is 0, set orientation to 0 rad
	else
		VCODE(12) = mod(target(stateindices(state, 6)), 360) * pi / 180.0;  % orientation (convert from (degrees) in target table to (rad))
    end

elseif target_type == 3

    % Handle rectangle target:
    VCODE(10) = target(stateindices(state, 4)) * 0.01;  % length (convert from (cm) in target table to (m))
    VCODE(11) = target(stateindices(state, 5)) * 0.01;  % height (convert from (cm) in target table to (m))

    if stateindices(state, 6) == 0
		VCODE(12) = 0;  % if orientation column is 0, set orientation to 0 rad
	else
		VCODE(12) = mod(target(stateindices(state, 6)), 360) * pi / 180.0;  % orientation (convert from (degrees) in target table to (rad))
    end
    
elseif target_type == 4

    % Handle line target:
    VCODE(10) = target(stateindices(state, 4)) * 0.01;  % line endpoint in x axis, relative to start (convert from (cm) in target table to (m))
    VCODE(11) = target(stateindices(state, 5)) * 0.01;  % line endpoint in y axis, relative to start (convert from (cm) in target table to (m))

elseif target_type == 5

    % Handle triangle target:
    VCODE(10) = target(stateindices(state, 4)) * 0.01;  % length (convert from (cm) in target table to (m))

    % If the height column is set to 0 then the triangle is automatically made equilateral, with the base length used as length
    % for all sides. If the height column is non-zero, separate values for height and peak offset are taken from the target table.
    if stateindices(state, 5) == 0
        VCODE(11) = sin(pi / 3.0) * VCODE(10);  % height for equilateral triangle
        VCODE(12) = 0;                          % peak offset for equilateral triangle
    else
        VCODE(11) = target(stateindices(state, 5)) * 0.01;  % height (convert from (cm) in target table to (m))
        VCODE(12) = target(stateindices(state, 6)) * 0.01;  % peak offset (convert from (cm) in target table to (m))
    end

    if stateindices(state, 7) == 0
        VCODE(13) = 0;  % if orientation column is 0, set orientation to 0 rad
    else
        VCODE(13) = mod(target(stateindices(state, 7)), 360) * pi / 180.0;  % orientation (convert from (degrees) in target table to (rad))
    end
end


% The colourshift function converts an "RRRGGGBBB" colour value to RRGBB (as an uint32).
function RRGGBBAA = colourshift(RRRGGGBBB)

blue = cast(mod(RRRGGGBBB, 1000), 'uint32');
green = cast(mod(RRRGGGBBB - blue, 1000000) / 1000, 'uint32');
red = cast((RRRGGGBBB - (green * 1000) - blue) / 1000000, 'uint32');

RRGGBBAA = bitshift(red, 16) + bitshift(green, 8) + blue;

== matlab function Custom Hand Feedback/Hand_Feedback_2_hands_or_mean/FeedFwdArm ==
  settings: fimath=|
      | fimath(...
      | 'RoundMode', 'floor',...
      | 'OverflowMode', 'wrap',...
      | 'ProductMode', 'KeepLSB', 'ProductWordLength', 32,...
      | 'SumMode', 'KeepLSB', 'SumWordLength', 32,...
      | 'CastBeforeSum', false)
  data: VCODES_in input double; num_cursors input double; VCODES_out output double; mean_hand_position input double
function VCODES_out  = fcn(VCODES_in, num_cursors, mean_hand_position)
%

VCODES_out = VCODES_in;     %default

if num_cursors == 1;
    %show ONLY dominant hand feedback, but show mean hand position
	VCODES_out(1,2)=1;
	VCODES_out(2,2)=0;

	VCODES_out(1,3)=mean_hand_position(1);		%target position in m 
	VCODES_out(1,4)=mean_hand_position(2);		%target position in m 
end
% ***************************************
